simulink model "chirp_waveform_generator"  (R2024a)
settings: Solver=VariableStepAuto  StartTime=0.0  StopTime=0.0005  RelTol=1e-3
undefined symbols (not defined in the file): AXI4, Lite
libraries: hdlBasic x32, hdlDSPIP x1, vmcUtilities x1
settings Model: Creator=ehtisham  LastModifiedBy=ehtisham

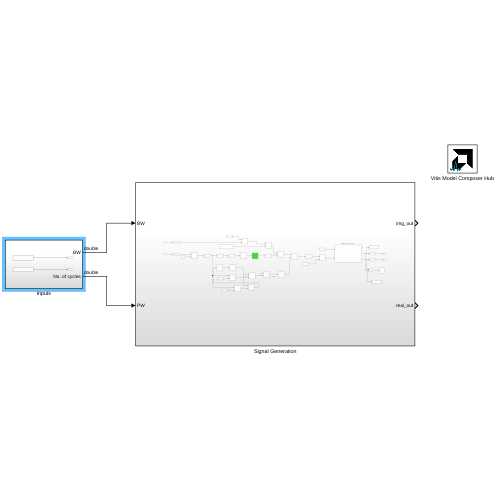
[thumbnail: Simulink's stored preview of the top-level diagram]
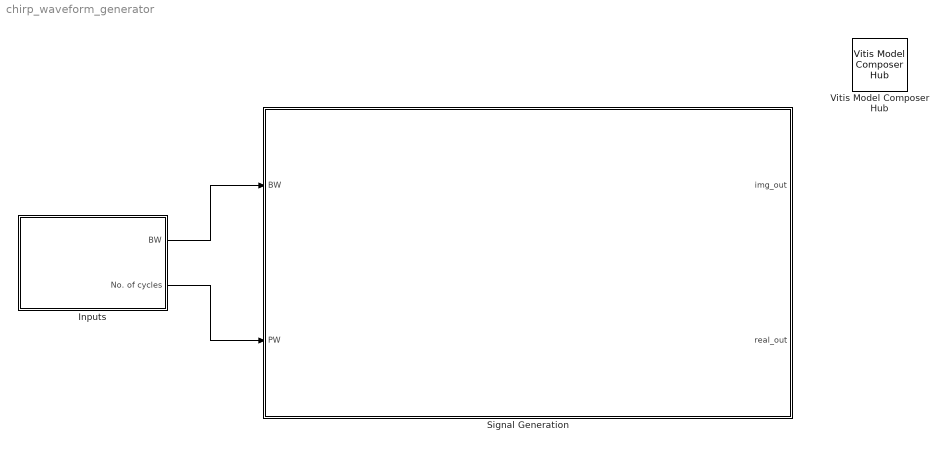
== system chirp_waveform_generator ==
  Inputs : Subsystem
  Signal Generation : Subsystem
  Vitis Model Composer Hub : vmcUtilities/Vitis Model Composer Hub  Tag=genX  CodeGeneration=off  SubsystemName=Signal Generation  CompilationType=HDLCompilation  SubsystemType=HDLNode  ExportTypeV2=IP Catalog  StartColumn=1  NumberOfColumns=1  TargetDirectory=/home/ehtisham/Desktop/Ehtisham/Practice/Model_composer/Signal_Generation/IP1  exportDesign=on  analyzeDesign=off  validateDesignOnHw=off  ExportType=AI Engines  IpVendor=xilinx.com  IpLibrary=hls  IpVersion=1.0  IpHWLanguage=Verilog  AieCompilerOptions={}  AieSimulatorOptions={}  CreateTestbench=on  TestbenchStackSize=10  RunRtlSim=off  RunCSim=off  RunAieSim=off  AieSimTimeout=50000  RunAieSimProfiling=off  LaunchVitisAnalyzer=off  PlotOutput=off  RunX86Sim=off  X86SimTimeout=10  GenHwImage=off  GenLibadfXo=off  GenHwValidationCode=off  PlatformType=Not Specified  HwSystemType=Baremetal  HwValidationTarget=hw  ProjDevice=Zynq UltraScale+ ZCU102 Evaluation Board (xczu9eg-ffvb1156-2-e)  ProjDevicePart=xczu9eg-ffvb1156-2-e  AIEType=None  SamplePeriod=-1  ClockFrequency=200  DataPathParallelism=1  xilinxfamily=zynquplus  part=xczu9eg  speed=-2-e  package=ffvb1156  directory=/home/ehtisham/Desktop/Ehtisham/Practice/Model_composer/Signal_Generation/IP1/ip/Signal_Generation/src  testbench=on  incr_netlist=off  synthesis_tool=Vivado  clock_wrapper=Clock Enables  dbl_ovrd=According to Block Masks  dcm_input_clock_period=10  sysclk_period=4  simulink_period=1/245760000  eval_field=0  IPInfoJsonString="{\"DUTSubsystemName\":\"Signal Generation\",\"HDLSubsystem\":{\"SubsystemName\":\"Signal_Generation\",\"IPName\":\"Chirp_Generator\",\"IPLibrary\":\"VMC\",\"IPVendor\":\"M Ehtisham\",\"IPVersion\":\"1.0\",\"TargetDirectory\":\"/home/ehtisham/Desktop/Ehtisham/Practice/Model_composer/Signal_Generation/IP1\",\"SubsystemDir\":\"/home/ehtisham/Desktop/Ehtisham/Practice/Model_composer/Signal_Generation/IP1/ip/Signal_Generation\",\"FreqHz\":\"250000000\"},\"SubsystemTag\":\"HDLNode\"}"  LogFileName=/home/ehtisham/Desktop/Ehtisham/Practice/Model_composer/Signal_Generation/IP1/model_composer.log  NThreads=4  IPConfigFile=/tmp/vmctmp-ehtisham/2407313/ipconfig.json
  wires:
  Inputs/1(BW) -> Signal Generation/1(BW)
  Inputs/2(No. of cycles) -> Signal Generation/2(PW)

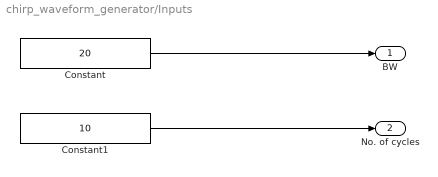
== system chirp_waveform_generator/Inputs ==
  Constant : Constant  Value=20
  Constant1 : Constant  Value=10
  BW : Outport
  No. of cycles : Outport  Port=2
  wires:
  Constant/1 -> BW/1
  Constant1/1 -> No. of cycles/1

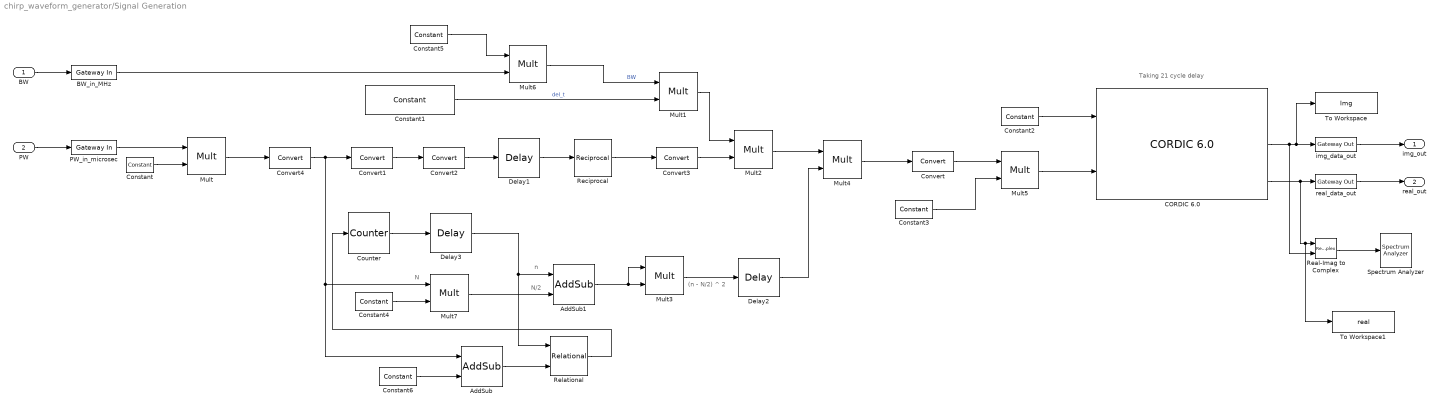
== system chirp_waveform_generator/Signal Generation ==
  note: Taking 21 cycle delay
  note: n
  note: N/2
  note: N
  note: (n - N/2) ^ 2
  BW : Inport
  PW : Inport  Port=2
  AddSub : hdlBasic/AddSub  mode=Subtraction  use_carryin=off  use_carryout=off  en=off  latency=0  precision=Full  arith_type=Unsigned  n_bits=16  bin_pt=14  quantization=Truncate  overflow=Wrap  use_behavioral_HDL=off  hw_selection=Fabric  pipelined=off  XmcBlockStatus=1  maskContainerNames=tabcontainer1  block_type=addsub  block_config=sysgen:Addsub_config
  AddSub1 : hdlBasic/AddSub  mode=Subtraction  use_carryin=off  use_carryout=off  en=off  latency=0  precision=Full  arith_type=Unsigned  n_bits=16  bin_pt=14  quantization=Truncate  overflow=Wrap  use_behavioral_HDL=off  hw_selection=Fabric  pipelined=off  XmcBlockStatus=1  maskContainerNames=tabcontainer1  block_type=addsub  block_config=sysgen:Addsub_config
  BW_in_MHz : hdlBasic/Gateway In  gui_display_data_type=Fixed-point  arith_type=Unsigned  n_bits=7  bin_pt=0  preci_type=Single  exp_width=8  frac_width=24  rows=1  columns=1  quantization="Round  (unbiased: +/- Inf)"  overflow=Saturate  period=1/245760000  UseAsADC=off  ADCChannel='1'  interface=AXI4-Lite  automatic_assignment=on  address_offset=hex2dec('00')  intf_name='signal_bw'  intf_description='This is the chirp BW. User have to enter BW value in MHz'  default_value=0  timing_constraint=None  locs_specified=off  LOCs={}  io_standard={}  inherit_from_input=off  hdl_port=on  XmcBlockStatus=1  maskContainerNames=group4  block_type=gatewayin  block_config=sysgen:gateway_in_config  block_width_w=590  block_height_w=620  block_width=640  block_height=850
  CORDIC 6.0 : hdlDSPIP/CORDIC 6.0   functional_selection=Sin_and_Cos  architectural_configuration=Parallel  pipelining_mode=Maximum  data_format=SignedFraction  phase_format=Radians  input_width=48  output_width=16  round_mode=Truncate  iterations=0  precision=0  compensation_scaling=No_Scale_Compensation  coarse_rotation=on  aclken=off  aresetn=off  out_tready=off  cartesian_has_tuser=off  cartesian_has_tlast=off  cartesian_tuser_width=1  phase_has_tuser=off  phase_has_tlast=off  phase_tuser_width=1  out_tlast_behv=Null  flow_control=NonBlocking  optimize_goal=Performance  trim_axipin_name=on  simulation_type=hybrid_sim  simulation_model=sysgen:cordic_v6_0  data_path_portlist={'s_axis_cartesian_tdata_imag', 's_axis_cartesian_tdata_real', 's_axis_phase_tdata_phase', 'm_axis_dout_tdata_imag', 'm_axis_dout_tdata_real', 'm_axis_dout_tdata_phase','m_axis_dout_tdata'}  ip_name=CORDIC  ip_version=6.0  dsptool_ready=true  ipcore_usecache=true  ipcore_useipmodelcache=true  wrapper_available=true  port_translation_map={ 'aclken' => 'en', 'aresetn' => 'rst' }  XmcBlockStatus=1  maskContainerNames=group15  block_type=cordic_v6_0  block_config=sysgen:rodinimport_config  block_width=800
  Constant : hdlBasic/Constant  const=245.76  gui_display_data_type=Fixed-point  arith_type=Unsigned  n_bits=12  bin_pt=4  preci_type=Single  exp_width=8  frac_width=24  explicit_period=off  period=1  XmcBlockStatus=1  maskContainerNames=tabcontainer1  block_type=constant  block_config=sysgen:Constant_config
  Constant1 : hdlBasic/Constant  const=1/245760000  gui_display_data_type=Fixed-point  arith_type=Unsigned  n_bits=40  bin_pt=39  preci_type=Single  exp_width=8  frac_width=24  explicit_period=on  period=1/245760000  XmcBlockStatus=1  maskContainerNames=tabcontainer1  block_type=constant  block_config=sysgen:Constant_config
  Constant2 : hdlBasic/Constant  const=1.0  gui_display_data_type=Boolean  arith_type=Boolean  n_bits=16  bin_pt=14  preci_type=Single  exp_width=8  frac_width=24  explicit_period=off  period=1  XmcBlockStatus=1  maskContainerNames=tabcontainer1  block_type=constant  block_config=sysgen:Constant_config
  Constant3 : hdlBasic/Constant  const=3.14  gui_display_data_type=Fixed-point  arith_type=Unsigned  n_bits=8  bin_pt=6  preci_type=Single  exp_width=8  frac_width=24  explicit_period=on  period=1/245760000  XmcBlockStatus=1  maskContainerNames=tabcontainer1  block_type=constant  block_config=sysgen:Constant_config
  Constant4 : hdlBasic/Constant  const=0.5  gui_display_data_type=Fixed-point  arith_type=Unsigned  n_bits=2  bin_pt=2  preci_type=Single  exp_width=8  frac_width=24  explicit_period=on  period=1/245760000  XmcBlockStatus=1  maskContainerNames=tabcontainer1  block_type=constant  block_config=sysgen:Constant_config
  Constant5 : hdlBasic/Constant  const=1000000  gui_display_data_type=Fixed-point  arith_type=Unsigned  n_bits=20  bin_pt=0  preci_type=Single  exp_width=8  frac_width=24  explicit_period=on  period=1/245760000  XmcBlockStatus=1  maskContainerNames=tabcontainer1  block_type=constant  block_config=sysgen:Constant_config
  Constant6 : hdlBasic/Constant  const=1.0  gui_display_data_type=Fixed-point  arith_type=Unsigned  n_bits=1  bin_pt=0  preci_type=Single  exp_width=8  frac_width=24  explicit_period=off  period=1  XmcBlockStatus=1  maskContainerNames=tabcontainer1  block_type=constant  block_config=sysgen:Constant_config
  Convert : hdlBasic/Convert  gui_display_data_type=Fixed-point  arith_type=Signed (2's comp)  n_bits=18  bin_pt=17  float_type=Single  exp_bits=8  fraction_bits=24  quantization=Truncate  overflow=Wrap  en=off  latency=1  pipeline=off  XmcBlockStatus=1  maskContainerNames=group2  block_type=convert  block_config=sysgen:Convert_config  block_width=595  block_height=885
  Convert1 : hdlBasic/Convert  gui_display_data_type=Fixed-point  arith_type=Signed (2's comp)  n_bits=17  bin_pt=0  float_type=Double  exp_bits=8  fraction_bits=24  quantization=Truncate  overflow=Wrap  en=off  latency=0  pipeline=off  XmcBlockStatus=1  maskContainerNames=group2  block_type=convert  block_config=sysgen:Convert_config  block_width=595  block_height=885
  Convert2 : hdlBasic/Convert  gui_display_data_type=Floating-point  arith_type=Floating-point  n_bits=17  bin_pt=0  float_type=Single  exp_bits=8  fraction_bits=24  quantization=Truncate  overflow=Wrap  en=off  latency=6  pipeline=off  XmcBlockStatus=1  maskContainerNames=group2  block_type=convert  block_config=sysgen:Convert_config  block_width=595  block_height=885
  Convert3 : hdlBasic/Convert  gui_display_data_type=Fixed-point  arith_type=Signed (2's comp)  n_bits=32  bin_pt=24  float_type=Double  exp_bits=8  fraction_bits=24  quantization="Round  (unbiased: +/- Inf)"  overflow=Saturate  en=off  latency=1  pipeline=off  XmcBlockStatus=1  maskContainerNames=group2  block_type=convert  block_config=sysgen:Convert_config  block_width=595  block_height=885
  Convert4 : hdlBasic/Convert  gui_display_data_type=Fixed-point  arith_type=Signed (2's comp)  n_bits=16  bin_pt=0  float_type=Double  exp_bits=8  fraction_bits=24  quantization="Round  (unbiased: Even Values)"  overflow=Wrap  en=off  latency=0  pipeline=off  XmcBlockStatus=1  maskContainerNames=group2  block_type=convert  block_config=sysgen:Convert_config  block_width=595  block_height=885
  Counter : hdlBasic/Counter  cnt_type=Free running  cnt_to=Inf  operation=Up  start_count=0  cnt_by_val=1  arith_type=Unsigned  n_bits=16  bin_pt=0  load_pin=off  rst=on  en=off  explicit_period=Explicit  period=1/245760000  use_behavioral_HDL=off  implementation=Fabric  XmcBlockStatus=1  maskContainerNames=group1  block_type=counter  block_config=sysgen:Counter_config  block_width=531  block_height=1023
  Delay1 : hdlBasic/Delay  rst=off  en=off  latency=0  reg_retiming=off  XmcBlockStatus=1  maskContainerNames=group1  block_type=delay  block_config=sysgen:Delay_config
  Delay2 : hdlBasic/Delay  rst=off  en=off  latency=2  reg_retiming=off  XmcBlockStatus=1  maskContainerNames=group1  block_type=delay  block_config=sysgen:Delay_config
  Delay3 : hdlBasic/Delay  rst=off  en=off  latency=3  reg_retiming=off  XmcBlockStatus=1  maskContainerNames=group1  block_type=delay  block_config=sysgen:Delay_config
  Mult : hdlBasic/Mult  precision=Full  arith_type="Signed  (2's comp)"  n_bits=16  bin_pt=14  quantization=Truncate  overflow=Wrap  en=off  latency=0  opt_float=off  fp_mult_usage=No Usage  use_behavioral_HDL=off  opt=Speed  use_embedded=on  optimum_pipeline=off  pipeline=on  use_rpm=on  placement_style=Triangular  XmcBlockStatus=1  maskContainerNames=group1  block_type=mult  block_config=sysgen:Mult_config  block_width=598  block_height=876
  Mult1 : hdlBasic/Mult  precision=Full  arith_type="Signed  (2's comp)"  n_bits=16  bin_pt=14  quantization=Truncate  overflow=Wrap  en=off  latency=9  opt_float=off  fp_mult_usage=No Usage  use_behavioral_HDL=off  opt=Speed  use_embedded=on  optimum_pipeline=on  pipeline=on  use_rpm=on  placement_style=Triangular  XmcBlockStatus=1  maskContainerNames=group1  block_type=mult  block_config=sysgen:Mult_config  block_width=598  block_height=876
  Mult2 : hdlBasic/Mult  precision=Full  arith_type="Signed  (2's comp)"  n_bits=16  bin_pt=14  quantization=Truncate  overflow=Wrap  en=off  latency=3  opt_float=off  fp_mult_usage=No Usage  use_behavioral_HDL=off  opt=Speed  use_embedded=on  optimum_pipeline=off  pipeline=on  use_rpm=on  placement_style=Triangular  XmcBlockStatus=1  maskContainerNames=group1  block_type=mult  block_config=sysgen:Mult_config  block_width=598  block_height=876
  Mult3 : hdlBasic/Mult  precision=Full  arith_type="Signed  (2's comp)"  n_bits=16  bin_pt=14  quantization=Truncate  overflow=Wrap  en=off  latency=10  opt_float=off  fp_mult_usage=No Usage  use_behavioral_HDL=off  opt=Speed  use_embedded=off  optimum_pipeline=on  pipeline=on  use_rpm=on  placement_style=Triangular  XmcBlockStatus=1  maskContainerNames=group1  block_type=mult  block_config=sysgen:Mult_config  block_width=598  block_height=876
  Mult4 : hdlBasic/Mult  precision=Full  arith_type="Signed  (2's comp)"  n_bits=48  bin_pt=45  quantization="Round  (unbiased: +/- Inf)"  overflow=Wrap  en=off  latency=2  opt_float=off  fp_mult_usage=No Usage  use_behavioral_HDL=off  opt=Speed  use_embedded=on  optimum_pipeline=off  pipeline=on  use_rpm=on  placement_style=Triangular  XmcBlockStatus=1  maskContainerNames=group1  block_type=mult  block_config=sysgen:Mult_config  block_width=598  block_height=876
  Mult5 : hdlBasic/Mult  precision=Full  arith_type="Signed  (2's comp)"  n_bits=48  bin_pt=45  quantization="Round  (unbiased: +/- Inf)"  overflow=Wrap  en=off  latency=0  opt_float=off  fp_mult_usage=No Usage  use_behavioral_HDL=off  opt=Speed  use_embedded=on  optimum_pipeline=off  pipeline=on  use_rpm=on  placement_style=Triangular  XmcBlockStatus=1  maskContainerNames=group1  block_type=mult  block_config=sysgen:Mult_config  block_width=598  block_height=876
  Mult6 : hdlBasic/Mult  precision=Full  arith_type="Signed  (2's comp)"  n_bits=16  bin_pt=14  quantization=Truncate  overflow=Wrap  en=off  latency=4  opt_float=off  fp_mult_usage=No Usage  use_behavioral_HDL=off  opt=Speed  use_embedded=on  optimum_pipeline=off  pipeline=on  use_rpm=on  placement_style=Triangular  XmcBlockStatus=1  maskContainerNames=group1  block_type=mult  block_config=sysgen:Mult_config  block_width=598  block_height=876
  Mult7 : hdlBasic/Mult  precision=Full  arith_type="Signed  (2's comp)"  n_bits=16  bin_pt=14  quantization=Truncate  overflow=Wrap  en=off  latency=3  opt_float=off  fp_mult_usage=No Usage  use_behavioral_HDL=off  opt=Speed  use_embedded=on  optimum_pipeline=off  pipeline=on  use_rpm=on  placement_style=Triangular  XmcBlockStatus=1  maskContainerNames=group1  block_type=mult  block_config=sysgen:Mult_config  block_width=598  block_height=876
  PW_in_microsec : hdlBasic/Gateway In  gui_display_data_type=Fixed-point  arith_type=Unsigned  n_bits=13  bin_pt=6  preci_type=Single  exp_width=8  frac_width=24  rows=1  columns=1  quantization="Round  (unbiased: +/- Inf)"  overflow=Saturate  period=1/245760000  UseAsADC=off  ADCChannel='1'  interface=AXI4-Lite  automatic_assignment=on  address_offset=hex2dec('00')  intf_name='pw_cycles'  intf_description='This is the PW cycles. We have to divide user PW with Fs to get the No. of cycles'  default_value=0  timing_constraint=None  locs_specified=off  LOCs={}  io_standard={}  inherit_from_input=off  hdl_port=on  XmcBlockStatus=1  maskContainerNames=group4  block_type=gatewayin  block_config=sysgen:gateway_in_config  block_width_w=590  block_height_w=620  block_width=640  block_height=850
  Real-Imag to Complex : RealImagToComplex
  Reciprocal : hdlBasic/Reciprocal  flow_control=NonBlocking  axi_optimize_goal=Resources  latency=6  has_a_tlast=off  has_a_tuser=off  en=off  has_result_tready=off  has_underflow=off  has_divide_by_zero=off  fpo_op_type=reciprocal  rate=1  has_b_tlast=false  has_b_tuser=false  result_tlast_behv=1  has_overflow=false  has_invalid_op=false  XmcBlockStatus=1  maskContainerNames=tabcontainer1  block_type=reciprocal  block_config=sysgen:FPOBlockDescriptor_config
  Relational : hdlBasic/Relational  mode=a=b  op_type=Bool  en=off  latency=0  XmcBlockStatus=1  maskContainerNames=tabcontainer1  block_type=relational  block_config=sysgen:Relational_config
  Spectrum Analyzer : SpectrumAnalyzer  WindowPosition=[560.000000,179.000000,800.000000,500.000000,]  Visible=on  ScopeFrameLocation=window  Span=245760000  StartFrequency=-122880000  StopFrequency=122880000  YLimits=[-44.44929046,18.76878932]  SelectedToolstripTab=spectrumAnalyzerToolstrip.channelMeasurementsTab
  To Workspace : ToWorkspace  VariableName=Img  SaveFormat=Timeseries  SampleTime=-1
  To Workspace1 : ToWorkspace  VariableName=real  SaveFormat=Timeseries  SampleTime=-1
  img_data_out : hdlBasic/Gateway Out  inherit_from_input=off  hdl_port=on  rows=1  columns=1  UseAsDAC=off  DACChannel='1'  interface=None  automatic_assignment=on  address_offset=hex2dec('00')  intf_name=''  intf_description=''  timing_constraint=None  locs_specified=off  LOCs={}  io_standard={}  XmcBlockStatus=1  maskContainerNames=group4  block_type=gatewayout  block_config=sysgen:gateway_out_config  block_width_w=590  block_height_w=620  block_width=620  block_height=750
  real_data_out : hdlBasic/Gateway Out  inherit_from_input=off  hdl_port=on  rows=1  columns=1  UseAsDAC=off  DACChannel='1'  interface=None  automatic_assignment=on  address_offset=hex2dec('00')  intf_name=''  intf_description=''  timing_constraint=None  locs_specified=off  LOCs={}  io_standard={}  XmcBlockStatus=1  maskContainerNames=group4  block_type=gatewayout  block_config=sysgen:gateway_out_config  block_width_w=590  block_height_w=620  block_width=620  block_height=750
  img_out : Outport
  real_out : Outport  Port=2
  wires:
  BW/1 -> BW_in_MHz/1
  PW/1 -> PW_in_microsec/1
  Constant1/1 -> Mult1/2  "del_t"
  Mult6/1 -> Mult1/1  "BW"
  Counter/1 -> Delay3/1
  Mult2/1 -> Mult4/1
  Mult4/1 -> Convert/1
  Constant2/1 -> CORDIC 6.0/1
  CORDIC 6.0/3 -> To Workspace1/1, Real-Imag to Complex/1, real_data_out/1
  CORDIC 6.0/2 -> To Workspace/1, img_data_out/1, Real-Imag to Complex/2
  img_data_out/1 -> img_out/1
  real_data_out/1 -> real_out/1
  BW_in_MHz/1 -> Mult6/2
  Convert/1 -> Mult5/1
  Constant3/1 -> Mult5/2
  Mult5/1 -> CORDIC 6.0/2
  Relational/1 -> Counter/1
  Constant5/1 -> Mult6/1
  AddSub/1 -> Relational/2
  Constant6/1 -> AddSub/2
  Mult1/1 -> Mult2/1
  PW_in_microsec/1 -> Mult/1
  Reciprocal/1 -> Convert3/1
  Convert1/1 -> Convert2/1
  Convert2/1 -> Delay1/1
  Convert3/1 -> Mult2/2
  Mult3/1 -> Delay2/1
  Delay1/1 -> Reciprocal/1
  Delay2/1 -> Mult4/2
  Constant4/1 -> Mult7/2
  Mult7/1 -> AddSub1/2
  Delay3/1 -> Relational/1, AddSub1/1
  AddSub1/1 -> Mult3/2, Mult3/1
  Real-Imag to Complex/1 -> Spectrum Analyzer/1
  Constant/1 -> Mult/2
  Mult/1 -> Convert4/1
  Convert4/1 -> AddSub/1, Mult7/1, Convert1/1
